simulink model "AMDSB_demodulador"  (Simulink 7.7)
settings: Solver=ode45  StartTime=0.0  StopTime=10.0  MaxStep=1e-2  RelTol=1e-3
values from neighbouring files (symbols this model uses):
  a = 1    [AMDSB_demodulador_main.m]    (also in AMDSB_nao_linear_main.m)
  b = 1    [AMDSB_demodulador_main.m]    (also in AMDSB_nao_linear_main.m)
  c = 1    [AMDSB_demodulador_main.m]    (also in AMDSB_nao_linear_main.m; Base_main.m = linspace(0,2,M); base_otima.m = p)
  Den = [1 1]    [AMDSB_demodulador_main.m]    (also in AMDSB_nao_linear_main.m; AMDSB_sincrono_main.m)
  Num = 1    [AMDSB_demodulador_main.m]    (also in AMDSB_nao_linear_main.m; AMDSB_sincrono_main.m)
undefined symbols (not defined in the file or in its folder): magnitude
settings Model: Creator=vparro  LastModifiedBy=vanderleiparro
settings DebuggingCC: StrictBusMsg=Warning

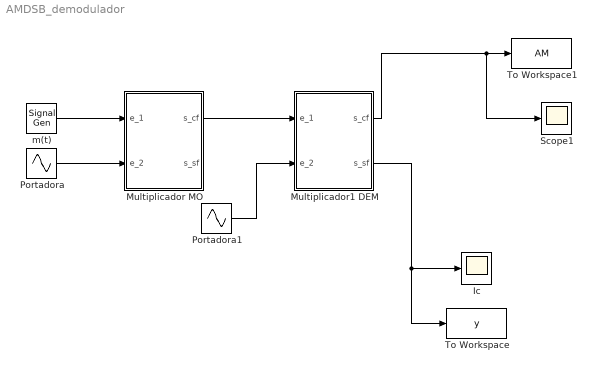
== system AMDSB_demodulador ==
  Ic : Scope
  Multiplicador MO : Subsystem
  Multiplicador1 DEM : Subsystem
  Portadora : Sin  Frequency=20*pi  SampleTime=0
  Portadora1 : Sin  Frequency=20*pi  SampleTime=0
  Scope1 : Scope
  To Workspace : ToWorkspace  VariableName=y  SampleTime=-1  SaveFormat=Array
  To Workspace1 : ToWorkspace  VariableName=AM  SampleTime=-1  SaveFormat=Array
  m(t) : SignalGenerator
  wires:
  Portadora/1 -> Multiplicador MO/2(e_2)
  m(t)/1 -> Multiplicador MO/1(e_1)
  Multiplicador MO/1(s_cf) -> Multiplicador1 DEM/1(e_1)
  Portadora1/1 -> Multiplicador1 DEM/2(e_2)
  Multiplicador1 DEM/1(s_cf) -> To Workspace1/1, Scope1/1
  Multiplicador1 DEM/2(s_sf) -> Ic/1, To Workspace/1

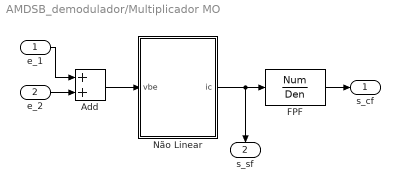
== system AMDSB_demodulador/Multiplicador MO ==
  e_1 : Inport
  e_2 : Inport  Port=2
  Add : Sum
  FPF : TransferFcn  Numerator=Num  Denominator=Den
  Não Linear : Subsystem
  s_cf : Outport
  s_sf : Outport  Port=2
  wires:
  Add/1 -> Não Linear/1(vbe)
  Não Linear/1(ic) -> FPF/1, s_sf/1
  e_1/1 -> Add/1
  FPF/1 -> s_cf/1
  e_2/1 -> Add/2

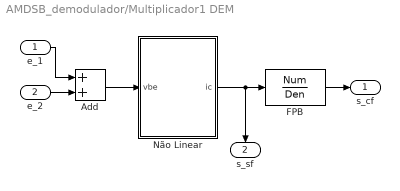
== system AMDSB_demodulador/Multiplicador1 DEM ==
  e_1 : Inport
  e_2 : Inport  Port=2
  Add : Sum
  FPB : TransferFcn  Numerator=Num  Denominator=Den
  Não Linear : Subsystem
  s_cf : Outport
  s_sf : Outport  Port=2
  wires:
  e_2/1 -> Add/2
  FPB/1 -> s_cf/1
  e_1/1 -> Add/1
  Não Linear/1(ic) -> s_sf/1, FPB/1
  Add/1 -> Não Linear/1(vbe)

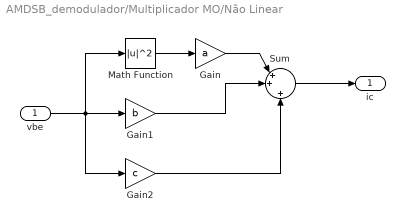
== system AMDSB_demodulador/Multiplicador MO/Não Linear ==
  vbe : Inport
  Gain : Gain  Gain=a
  Gain1 : Gain  Gain=b
  Gain2 : Gain  Gain=c
  Math Function : Math  Operator=magnitude^2  SaturateOnIntegerOverflow=on
  Sum : Sum  Inputs=|++|+
  ic : Outport
  wires:
  Math Function/1 -> Gain/1
  Gain/1 -> Sum/1
  Gain1/1 -> Sum/2
  Gain2/1 -> Sum/3
  vbe/1 -> Gain1/1, Math Function/1, Gain2/1
  Sum/1 -> ic/1

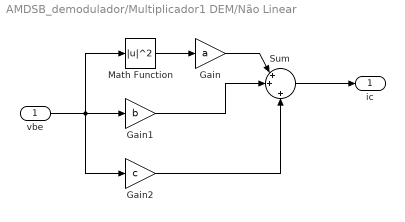
== system AMDSB_demodulador/Multiplicador1 DEM/Não Linear ==
  vbe : Inport
  Gain : Gain  Gain=a
  Gain1 : Gain  Gain=b
  Gain2 : Gain  Gain=c
  Math Function : Math  Operator=magnitude^2  SaturateOnIntegerOverflow=on
  Sum : Sum  Inputs=|++|+
  ic : Outport
  wires:
  Sum/1 -> ic/1
  vbe/1 -> Gain2/1, Math Function/1, Gain1/1
  Gain2/1 -> Sum/3
  Gain1/1 -> Sum/2
  Gain/1 -> Sum/1
  Math Function/1 -> Gain/1
